simulink model "signal_filter"  (R2025b)
settings: Solver=FixedStepDiscrete  StartTime=0.0  StopTime=1  FixedStep=Ts  RelTol=1e-3
model workspace (MAT data in the model file):
  Ts = Simulink.Parameter
  Ts.Value = 0.0001
  Ts.Complexity = 'real'
  Ts.Dimensions = [1 1]
  Ts.CoderInfo.StorageClass = 'SimulinkGlobal'
  Ts.Description = 'Sample period [s] (= LabVIEW loop period)'
  Ts.DataType = 'auto'
  filter_mode = Simulink.Parameter
  filter_mode.Value = 4
  filter_mode.Complexity = 'real'
  filter_mode.Dimensions = [1 1]
  filter_mode.CoderInfo.StorageClass = 'SimulinkGlobal'
  filter_mode.Description = '0 bypass,1 LPF1,2 Butter2,3 MovAvg,4 Kalman,5 Particle'
  filter_mode.DataType = 'auto'
  lpf_fc = Simulink.Parameter
  lpf_fc.Value = 200
  lpf_fc.Complexity = 'real'
  lpf_fc.Dimensions = [1 1]
  lpf_fc.CoderInfo.StorageClass = 'SimulinkGlobal'
  lpf_fc.Description = 'LPF cutoff [Hz] (modes 1,2)'
  lpf_fc.DataType = 'auto'
  ma_len = Simulink.Parameter
  ma_len.Value = 20
  ma_len.Complexity = 'real'
  ma_len.Dimensions = [1 1]
  ma_len.CoderInfo.StorageClass = 'SimulinkGlobal'
  ma_len.Description = 'Moving-average window [samples] (mode 3, max 1000)'
  ma_len.DataType = 'auto'
  meas_r = Simulink.Parameter
  meas_r.Value = 0.04
  meas_r.Complexity = 'real'
  meas_r.Dimensions = [1 1]
  meas_r.CoderInfo.StorageClass = 'SimulinkGlobal'
  meas_r.Description = 'Measurement noise variance (modes 4,5)'
  meas_r.DataType = 'auto'
  pf_N = Simulink.Parameter
  pf_N.Value = 200
  pf_N.Complexity = 'real'
  pf_N.Dimensions = [1 1]
  pf_N.CoderInfo.StorageClass = 'SimulinkGlobal'
  pf_N.Description = 'Particle count (mode 5, max 1000)'
  pf_N.DataType = 'auto'
  proc_q = Simulink.Parameter
  proc_q.Value = 100000
  proc_q.Complexity = 'real'
  proc_q.Dimensions = [1 1]
  proc_q.CoderInfo.StorageClass = 'SimulinkGlobal'
  proc_q.Description = 'Process noise density (modes 4,5)'
  proc_q.DataType = 'auto'
values from neighbouring files (symbols this model uses):
  Ts = max(Ts, 1e-6)    [signal_filter_core.m]
settings Model: Creator=REM2  LastModifiedBy=REM2
settings OptimizationCC: DefaultParameterBehavior=Inlined

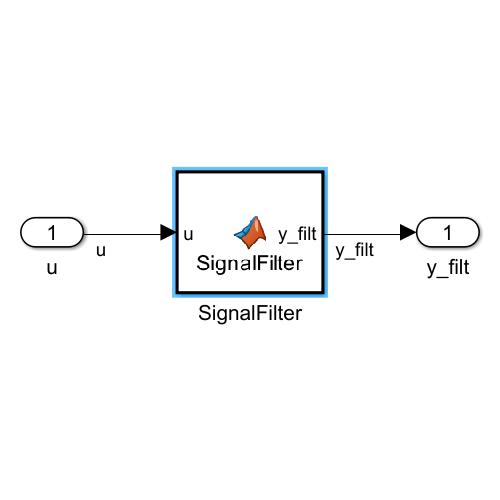
[thumbnail: Simulink's stored preview of the top-level diagram]
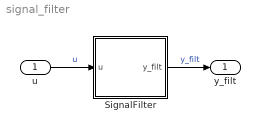
== system signal_filter ==
  u : Inport
  SignalFilter : MATLAB Function  TreatAsAtomicUnit=on
  y_filt : Outport
  wires:
  SignalFilter/1(y_filt) -> y_filt/1  "y_filt"
  u/1 -> SignalFilter/1(u)  "u"

== matlab function signal_filter/SignalFilter ==
  data: u input; y_filt output; filter_mode parameter; Ts parameter; lpf_fc parameter; ma_len parameter; proc_q parameter; meas_r parameter; pf_N parameter
function y_filt = SignalFilter(u, filter_mode, Ts, lpf_fc, ma_len, proc_q, meas_r, pf_N)
% filter_mode: 0 bypass, 1 LPF1, 2 Butterworth2, 3 moving avg, 4 Kalman, 5 particle.
% All inputs except u are tunable model-workspace parameters.
y_filt = signal_filter_core(u, filter_mode, Ts, lpf_fc, ma_len, proc_q, meas_r, pf_N);
